simulink model "projectile"  (R2026a)
settings: Solver=FixedStepAuto  StopTime=11.1  FixedStep=1/10
values from neighbouring files (symbols this model uses):
  g = 9.81    [parametres_TP_projectile.m]
  pos_x0 = 0    [Projectile_parameters.m]    (also in parametres_TP_projectile.m)
  pos_y0 = 0    [Projectile_parameters.m]    (also in parametres_TP_projectile.m)
  vit_x0 = vit0*cos(theta)    [Projectile_parameters.m]    (also in parametres_TP_projectile.m)
  vit_y0 = vit0*sin(theta)    [Projectile_parameters.m]    (also in parametres_TP_projectile.m)
settings Model: Creator=lulu1  LastModifiedBy=lulu1

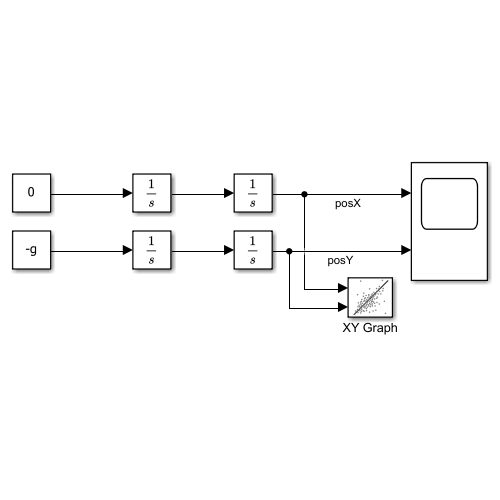
[thumbnail: Simulink's stored preview of the top-level diagram]
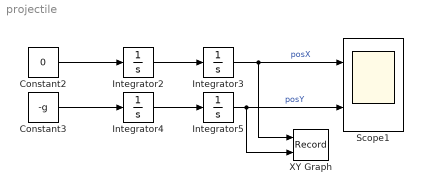
== system projectile ==
  Constant2 : Constant  Value=0
  Constant3 : Constant  Value=-g
  Integrator2 : Integrator  InitialCondition=vit_x0
  Integrator3 : Integrator  InitialCondition=pos_x0
  Integrator4 : Integrator  InitialCondition=vit_y0
  Integrator5 : Integrator  InitialCondition=pos_y0
  Scope1 : Scope  NumInputPorts=2
      settings: ActiveDisplayYMinimum=-81.392222081391282  ActiveDisplayYMaximum=732.52999873252168
  XY Graph : Record  NumPorts=2.0  FileSettingsInternal="{\"entries\":[{\"content\":{\"excelSettings\":{\"content\":{},\"type\":\"Streamout.ExcelSettings\"},\"parquetSettings\":{\"content\":{},\"type\":\"Streamout.ParquetSettings\"}},\"type\":\"Streamout.FileSettingStorage\",\"uuid\":\"\"}],\"packageUris\":[\"http:\\/\\/schema.mathworks.com\\/mf0\\/streamout_blocks\\/R2020a\"],\"version\":\"1.0\"}"  FrameSettings=[0, 0]  Layout=[1 1]  SignalsInternal="{\"entries\":[{\"content\":{\"signals\":[{\"content\":{\"blockPath\":[],\"dimensions\":[1],\"domain\":\"\",\"lineColor\":\"#a2142f\",\"plots\":[ 1 ],\"port\":1,\"sid\":[\"\"],\"signalID\":1,\"signalName\":\"posX\"},\"type\":\"RecordBlkView.Signal\",\"uuid\":\"\"},{\"content\":{\"blockPath\":[],\"dimensions\":[1],\"domain\":\"\",\"lineColor\":\"#139fff\",\"plots\":[ 1 ],\"port\":2,\"sid\":[\"\"],\"signalID\":2,\"signalName\":\"posY\"},\"type\":\"RecordBlkView.Signal\",\"uuid\":\"\"}]},\"type\":\"RecordBlkView.InputSignals\",\"uuid\":\"\"}],\"packageUris\":[\"http:\\/\\/schema.mathworks.com\\/mf0\\/streamout_blocks\\/R2020a\"],\"version\":\"1.0\"}"  VisualizationBindings="{\"xyplotplugin\":{\"info\":[{\"series\":[{\"bindingParametersList\":[{\"parameter\":\"X-Axis\",\"signalID\":1,\"signalName\":\"posX\"},{\"parameter\":\"Y-Axis\",\"signalID\":2,\"signalName\":\"posY\"}],\"seriesID\":0}],\"subplotID\":1}]}}"  CompatibilityTag=XY
  wires:
  Integrator2/1 -> Integrator3/1
  Constant2/1 -> Integrator2/1
  Integrator3/1 -> XY Graph/1, Scope1/1  "posX"
  Integrator4/1 -> Integrator5/1
  Constant3/1 -> Integrator4/1
  Integrator5/1 -> XY Graph/2, Scope1/2  "posY"
